simulink library "mssSimulink"  (R2024a)
settings: Solver=ode45  StartTime=0.0  StopTime=10.0  RelTol=1e-3
undefined symbols (not defined in the file): ABC, CN_data, CX_data, CY_data, D, G, Hoerner, K_supply, kt2ms, MA, magnitude, MRB, pathlength, RAO_Amp, RAO_Dir, RAO_Freq, RAO_Phase, RAO_Vel, RAO_yaw_back, RAO_yaw_quant, RAO_yaw_quantization_flag, rho_a, slcm, T_supply, table, vessel, vesselABC
libraries: $bdroot x99, simulink x13
(part 4 of 9)

== system mssSimulink/Modelling/Environmental Loads ==
  Force RAO : Subsystem  mask(Force RAO){RAO_Freq=vessel.forceRAO.w, RAO_Dir=vessel.headings, RAO_Vel=vessel.velocities, RAO_Amp=vessel.forceRAO.amp, RAO_Phase=vessel.forceRAO.phase, RAO_add_omega_0=on, RAO_add_omega_inf=on, RAO_yaw_quantization_flag=on, RAO_yaw_quant=10*pi/180, RAO_yaw_back=2.5*pi/180, RAO_speed_backlash_flag=on, RAO_speed_back=1, RAO_smoothing_flag=on}
      mask prompts: RAO_Freq "Vector of frequencies RAO_Freq (rad/s)"; RAO_Dir "Vector of directions RAO_Dir (rad)"; RAO_Vel "Vector of velocities RAO_Vel (m/s)"; RAO_Amp "6DOF Cell array with tables of Amplitudes RAO_Amp"; RAO_Phase "6DOF Cell array with tables of Phases RAO_Phase (rad)"; RAO_add_omega_0 "Add asymptotic RAO values for omega = 0"; RAO_add_omega_inf "Add asymptotic RAO values for omega = inf"; RAO_yaw_quantization_flag "LF estimator for yaw angle table lookup (backlash and quantization)"; RAO_yaw_quant "LF yaw angle quantization interval [rad]"; RAO_yaw_back "LF yaw angle backlash width [rad] (typically 1/4 of the quantization interval)"; RAO_speed_backlash_flag "Speed lookup backlash (avoid rapid speed data switching)"; RAO_speed_back "Speed backlash widht [m/s]"; RAO_smoothing_flag "Smooth the output to avoid switching transients due to table lookup"
      mask help:
      | Calculate the 6 degrees-of-freedom (DOF) wave-frequency excitation forces Tau_WF for a vessel from its Force Response Amplitude Operators (Force RAOs) and a sea state defined by a set of harmonic waves. The block takes the "Waves" bus from the MSS Waves block as input, as well as the vessel low-frequency (LF) motion in terms of the generalized position vector eta_LF and mean surge velocity U. See help for details.
      |
      | Copyright (C) NTNU 2005
      | Author: Oyvind N. Smogeli, 2005-05-03
      mask init:
      | % Add a second velocity if only one is given in order to avoid run-time errors in the table lookup blocks
      | if length(RAO_Vel) == 1
      | 
      | 	if RAO_Vel == 0 % Add a second identical data set for V = 5 m/s
      | 		RAO_Vel(2) = 5;
      | 	else % Add a second identical data set for V = 0 m/s
      | 		RAO_Vel = [0 RAO_Vel];
      | 	end
      | 
      | 	for dofno = 1:6
      | 		RAO_Amp{dofno}(:,:,2) = RAO_Amp{dofno}(:,:,1);
      | 		RAO_Phase{dofno}(:,:,2) = RAO_Phase{dofno}(:,:,1);
      | 	end
      | 
      | end
      | 
      | % Add RAO values for zero frequency: use values for lowest given frequency
      | if RAO_add_omega_0 > 0
      | 	
      | 	if min(RAO_Freq) > 0
      | 				
      | 		RAO_Freq = [0 RAO_Freq];
      | 		
      | 		for dofno = 1:6
      | 			RAO_Amp{dofno} = [RAO_Amp{dofno}(1,:,:); RAO_Amp{dofno}];
      | 			RAO_Phase{dofno} = [RAO_Phase{dofno}(1,:,:); RAO_Phase{dofno}];
      | 		end
      | 	
      | 	end
      | 	
      | end
      | 
      | % Add RAO values for high frequency: use values for highest given frequency
      | maxfreq = 100;
      | if RAO_add_omega_inf > 0
      | 
      | 	if max(RAO_Freq) < maxfreq
      | 			
      | 		newfreq = 2*max(RAO_Freq) - RAO_Freq(length(RAO_Freq)-1);
      | 		
      | 		RAO_Freq = [RAO_Freq newfreq maxfreq];
      | 		
      | 		for dofno = 1:6
      | 			RAO_Amp{dofno} = [RAO_Amp{dofno} ; zeros(2, length(RAO_Dir), length(RAO_Vel))];
      | 			RAO_Phase{dofno} = [RAO_Phase{dofno} ; zeros(2, length(RAO_Dir), length(RAO_Vel))];
      | 		end
      | 		
      | 	end
      | 
      | end
      mask Help:
      | <b>Part of the Marine Systems Simulator: MSS</b><br>
      | <br>
      | Calculate the 6 degrees-of-freedom (DOF) wave-frequency excitation forces Tau_WF
      | for a vessel from its Force Response Amplitude Operators (Force RAOs) and a sea
      | state defined by a set of harmonic waves. The block takes the &quot;Waves&quot; bus from
      | the MSS Waves block as input, as well as the vessel low-frequency (LF) motion in
      | terms of the generalized position vector eta_LF and mean surge velocity U.<p>The Force RAOs are defined in terms of a
      | vector of frequencies (RAO_Freq), a vector of directions (RAO_Dir), a vector of
      | velocities (RAO_Dir), a 6DOF cell array of 3D matrices with amplitudes
      | (RAO_Amp), and a 6DOF cell array of 3D matrices with phases (RAO_Phase), which
      | are all input in the block mask. The first dimension of the 3D matrices
      | corresponds to the frequencies, the second to the directions, and the third to
      | the velocities, such that e.g. the amplitude amp in heave (DOF #3) for frequency
      | number n_f, direction number n_d and velocity number n_v can be found from a =
      | RAO_Amp{3}(n_f, n_d, n_v).</p>
      | <p><b>Inputs:</b></p>
      | <p>Waves:&nbsp;&nbsp;&nbsp;&nbsp;&nbsp;&nbsp;&nbsp;&nbsp;&nbsp;&nbsp;&nbsp; Bus
      | containing the following signals<br>
      | &nbsp;&nbsp;&nbsp; Zeta_a:&nbsp;&nbsp;&nbsp;&nbsp;&nbsp;&nbsp;&nbsp; Vector of harmonic wave amplitudes [m]<br>
      | &nbsp;&nbsp;&nbsp; Omega:&nbsp;&nbsp;&nbsp;&nbsp;&nbsp;&nbsp; Vector of harmonic wave frequencies [rad/s]<br>
      | &nbsp;&nbsp;&nbsp; Phase:&nbsp;&nbsp;&nbsp;&nbsp;&nbsp;&nbsp;&nbsp;&nbsp; Vector of harmonic wave phases (random) [rad]<br>
      | &nbsp;&nbsp;&nbsp; Wavenum:&nbsp;&nbsp;&nbsp; Vector of harmonic wave numbers [1/m]<br>
      | &nbsp;&nbsp;&nbsp; Psi:&nbsp;&nbsp;&nbsp;&nbsp;&nbsp;&nbsp;&nbsp;&nbsp;&nbsp;&nbsp;&nbsp;&nbsp;&nbsp; Vector of harmonic wave directions [rad]</p>
      | <p>eta_LF:&nbsp;&nbsp;&nbsp;&nbsp;&nbsp;&nbsp;&nbsp;&nbsp;&nbsp;&nbsp;&nbsp;
      | Generalized 6DOF n-frame low-frequency position vector [x (m), y (m), z (m),
      | theta (rad), phi (rad), psi (rad)]<br>
      | U:&nbsp;&nbsp;&nbsp;&nbsp;&nbsp;&nbsp;&nbsp;&nbsp;&nbsp;&nbsp;&nbsp;&nbsp;&nbsp;&nbsp;&nbsp;&nbsp;&nbsp;&nbsp;&nbsp;
      | Low-frequency (mean) surge velocity&nbsp; [m/s]</p>
      | <p><b>Outputs:</b></p>
      | <p>tau_WF:&nbsp;&nbsp;&nbsp;&nbsp;&nbsp;&nbsp;&nbsp;&nbsp;&nbsp; Generalized
      | 6DOF h-frame force vector [X (N), Y (N), Z (N), K (Nm), M (Nm), N (Nm)]</p>
      | <p><b>Model validity:</b></p>
      | <p>The validity of the block is dependent on the validity of the given
      | RAO data set.</p>
      | <p>A proper RAO to be used with this block should contain at least 1 velocity, 5
      | directions (e.g. 0, 45, 90, 135 and 180 degrees) and 10-20 frequencies, for all
      | 6 DOF (surge, sway, heave, roll, pitch, yaw).</p>
      | <p>The block performs linear interpolation in frequencies and directions, and
      | uses the data set for the velocity closest to the input velocity (i.e. 'nearest'
      | interpolation in velocity). If the block recieves an input wave frequency or relative
      | wave direction outside the span of the data vectors RAO_Freq or RAO_Dir
      | respectively, the simulation stops and an error is returned. This means that a well-defined
      | RAO must contain data for both 0 and 180 degrees, and for frequencies covering
      | the desired range of wave frequencies. If desired, asymptotic values can be
      | automatically added for zero and infinity frequency to avoid runtime errors if
      | the wave freqeuncy exceeds the values in RAO_Freq (see checkboxes in the mask). </p>
      | <p>IMPORTANT NOTE: The RAO theory upon which this block is based is in reality
      | only valid when the vessel low-frequency (h-frame) motion is a constant surge
      | velocity only, and the vessel is performing wave-frequency oscillations about
      | the steadily translating h-frame.This means that the outputs from the block when
      | manoeuvering -- i.e. changing the surge velocity and/or yaw angle -- must be
      | interpreted with some care. A jump in the output must be expected when changing
      | between two velocity data sets, and frequency warping expected when changing the
      | yaw angle (due to interpolation in the phase). It is therefore recommended to
      | use backlash on the input velocity to avoid transient switching, and a quantized
      | yaw angle with backlash. The latter will lead to jump in the ouput when the yaw
      | angle changes from one quantized value to another, but will give better results
      | when keeping within one quantizer interval. The quantized yaw angle with
      | backlash and velocity with backlash are available as options via checkboxes in
      | the mask. If either of these are activated, proper values for the yaw
      | quantization interval, yaw backlash width, and the the speed backlash width
      | respectively must be set. Typical values could be a yaw quantization interval of
      | 5 degrees, yaw backlash width of 1/4-1/5 of the quantization interval, and speed
      | backlash width of 1 m/s. To avoid the most rapid transients when switching
      | between data sets, output smoothing is available as an option in the mask. If
      | this is enabled, the output during a transent is rate limited according to the
      | fastest recorded signal rate during normal operation.</p>
      | <p><b>Example mask input:</b></p><p>
      | As an example, the format of the mask input for 2 velocities, 3 directions and 5
      | frequencies is as follows:<p>RAO_Freq = [f1 f2 f3 f4 f5]<br>
      | RAO_Dir = [d1 d2 d3]<br>
      | RAO_Vel = [v1 v2]<p>Surge:<br>
      | RAO_Amp{1}(:,:,1)&nbsp; = [a1_111 a1_121 a1_131; a1_211 a1_221 a1_231; a1_311
      | a1_321 a1_331; a1_411 a1_421 a1_431; a1_511 a1_521 a1_531]<br>
      | RAO_Amp{1}(:,:,2)&nbsp; = [a1_112 a1_122 a1_132; a1_212 a1_222 a1_232; a1_312
      | a1_322 a1_332; a1_412 a1_422 a1_432; a1_512 a1_522 a1_532]<br>
      | RAO_Phase{1}(:,:,1) = [p1_111 p1_121 p1_131; p1_211 p1_221 p1_231; p1_311 p1_321
      | p1_331; p1_411 p1_421 p1_431; p1_511 p1_521 p1_531]<br>
      | RAO_Phase{1}(:,:,2) = [p1_112 p1_122 p1_132; p1_212 p1_222 p1_232; p1_312 p1_322
      | p1_332; p1_412 p1_422 p1_432; p1_512 p1_522 p1_532]<p>Sway:<br>
      | RAO_Amp{2}(:,:,1)&nbsp; = [a2_111 a2_121 a2_131; a2_211 a2_221 a2_231; a2_311
      | a2_321 a2_331; a2_411 a2_421 a2_431; a2_511 a2_521 a2_531]<br>
      | RAO_Amp{2}(:,:,2)&nbsp; = [a2_112 a2_122 a2_132; a2_212 a2_222 a2_232; a2_312
      | a2_322 a2_332; a2_412 a2_422 a2_432; a2_512 a2_522 a2_532]<br>
      | RAO_Phase{2}(:,:,1) = [p2_111 p2_121 p2_131; p2_211 p2_221 p2_231; p2_311 p2_321
      | p2_331; p2_411 p2_421 p2_431; p2_511 p2_521 p2_531]<br>
      | RAO_Phase{2}(:,:,2) = [p2_112 p2_122 p2_132; p2_212 p2_222 p2_232; p2_312 p2_322
      | p2_332; p2_412 p2_422 p2_432; p2_512 p2_522 p2_532]<p>...<p>Yaw:<br>
      | RAO_Amp{6}(:,:,1)&nbsp; = [a6_111 a6_121 a6_131; a6_211 a6_221 a6_231; a6_311
      | a6_321 a6_331; a6_411 a6_421 a6_431; a6_511 a6_521 a6_531]<br>
      | RAO_Amp{6}(:,:,2)&nbsp; = [a6_112 a6_122 a6_132; a6_212 a6_222 a6_232; a6_312
      | a6_322 a6_332; a6_412 a6_422 a6_432; a6_512 a6_522 a6_532]<br>
      | RAO_Phase{6}(:,:,1) = [p6_111 p6_121 p6_131; p6_211 p6_221 p6_231; p6_311 p6_321
      | p6_331; p6_411 p6_421 p6_431; p6_511 p6_521 p6_531]<br>
      | RAO_Phase{6}(:,:,2) = [p6_112 p6_122 p6_132; p6_212 p6_222 p6_232; p6_312 p6_322
      | p6_332; p6_412 p6_422 p6_432; p6_512 p6_522 p6_532]<p>where now for example the
      | amplitude and phase in sway (DOF 2) for frequency f5, direction d3 and velocity
      | v1 are given by RAO_Amp{2}(5,3,1) = a2_531 and RAO_Phase{2}(5,3,1) = p2_531.<p>
      | <b>Copyright (C) NTNU 2005</b></p>
      | <p><b>Author:</b> Oyvind N. Smogeli, 2005-05-03</p>
  Motion RAO : Subsystem  mask(Motion RAO){RAO_Freq=vessel.motionRAO.w, RAO_Dir=vessel.headings, RAO_Vel=vessel.velocities, RAO_Amp=vessel.motionRAO.amp, RAO_Phase=vessel.motionRAO.phase, RAO_add_omega_0=on, RAO_add_omega_inf=on, RAO_yaw_quantization_flag=off, RAO_yaw_quant=10*pi/180, RAO_yaw_back=2.5*pi/180, RAO_speed_backlash_flag=off, RAO_speed_back=2, RAO_smoothing_flag=on}
      mask prompts: RAO_Freq "Vector of frequencies RAO_Freq (rad/s)"; RAO_Dir "Vector of directions RAO_Dir (rad)"; RAO_Vel "Vector of velocities RAO_Vel (m/s)"; RAO_Amp "6DOF Cell array with tables of Amplitudes RAO_Amp"; RAO_Phase "6DOF Cell array with tables of Phases RAO_Phase (rad)"; RAO_add_omega_0 "Add asymptotic RAO values for omega = 0"; RAO_add_omega_inf "Add asymptotic RAO values for omega = inf"; RAO_yaw_quantization_flag "LF estimator for yaw angle table lookup (backlash and quantization)"; RAO_yaw_quant "LF yaw angle quantization interval [rad]"; RAO_yaw_back "LF yaw angle backlash width [rad] (typically 1/4 of the quantization interval)"; RAO_speed_backlash_flag "Speed lookup backlash (avoid rapid speed data switching)"; RAO_speed_back "Speed backlash widht [m/s]"; RAO_smoothing_flag "Smooth the output to avoid switching transients due to table lookup"
      mask help:
      | Calculate the wave-frequency motion of a vessel in 6 degrees-of-freedom (DOF) from its Motion Response Amplitude Operators (Motion RAOs) and a sea state defined by a set of harmonic waves. The block takes the "Waves" bus from the MSS Waves block as input, as well as the vessel low-frequency (LF) motion in terms of the generalized position vector eta_LF and mean surge velocity U. See help for details.
      |
      | Copyright (C) NTNU 2005
      | Author: Oyvind N. Smogeli, 2005-05-03
      mask init: same as mssSimulink/Modelling/Environmental Loads/Force RAO
      mask Help:
      | <b>Part of the Marine Systems Simulator: MSS</b><br>
      | <br>
      | Calculate the wave-frequency motion of a vessel in 6 degrees-of-freedom (DOF)
      | from its Motion Response Amplitude Operators (Motion RAOs) and a sea state
      | defined by a set of harmonic waves. The block takes the &quot;Waves&quot; bus from the MSS
      | Waves block as input, as well as the vessel low-frequency (LF) motion in terms
      | of the generalized position vector Eta_LF and surge velocity U.<p>
      | The Motion RAOs are defined in terms of a vector of frequencies (RAO_Freq), a
      | vector of directions (RAO_Dir), a vector of velocities (RAO_Dir), a 6DOF cell
      | array of 3D matrices with amplitudes (RAO_Amp), and a 6DOF cell array of 3D
      | matrices with phases (RAO_Phase), which are all input in the block mask. The
      | first dimension of the 3D matrices corresponds to the frequencies, the second to
      | the directions, and the third to the velocities, such that e.g. the amplitude
      | amp in heave (DOF #3) for frequency number n_f, direction number n_d and
      | velocity number n_v can be found from a = RAO_Amp{3}(n_f, n_d, n_v). </p>
      | <p><b>Inputs:</b></p>
      | <p>Waves:&nbsp;&nbsp;&nbsp;&nbsp;&nbsp;&nbsp;&nbsp;&nbsp;&nbsp;&nbsp;&nbsp; Bus
      | containing the following signals<br>
      | &nbsp;&nbsp;&nbsp; Zeta_a:&nbsp;&nbsp;&nbsp;&nbsp;&nbsp;&nbsp;&nbsp; Vector of harmonic wave amplitudes [m]<br>
      | &nbsp;&nbsp;&nbsp; Omega:&nbsp;&nbsp;&nbsp;&nbsp;&nbsp;&nbsp; Vector of harmonic wave frequencies [rad/s]<br>
      | &nbsp;&nbsp;&nbsp; Phase:&nbsp;&nbsp;&nbsp;&nbsp;&nbsp;&nbsp;&nbsp;&nbsp; Vector of harmonic wave phases (random) [rad]<br>
      | &nbsp;&nbsp;&nbsp; Wavenum:&nbsp;&nbsp;&nbsp; Vector of harmonic wave numbers [1/m]<br>
      | &nbsp;&nbsp;&nbsp; Psi:&nbsp;&nbsp;&nbsp;&nbsp;&nbsp;&nbsp;&nbsp;&nbsp;&nbsp;&nbsp;&nbsp;&nbsp;&nbsp; Vector of harmonic wave directions [rad]</p>
      | <p>eta_LF:&nbsp;&nbsp;&nbsp;&nbsp;&nbsp;&nbsp;&nbsp;&nbsp;&nbsp;&nbsp;&nbsp;
      | Generalized 6DOF n-frame low-frequency position vector [x (m), y (m), z (m),
      | theta (rad), phi (rad), psi (rad)]<br>
      | U:&nbsp;&nbsp;&nbsp;&nbsp;&nbsp;&nbsp;&nbsp;&nbsp;&nbsp;&nbsp;&nbsp;&nbsp;&nbsp;&nbsp;&nbsp;&nbsp;&nbsp;&nbsp;&nbsp;
      | Low-frequency (mean) surge velocity&nbsp; [m/s]</p>
      | <p><b>Outputs:</b></p>
      | <p>eta_WF:&nbsp;&nbsp;&nbsp;&nbsp;&nbsp;&nbsp;&nbsp;&nbsp;&nbsp; Generalized
      | 6DOF n-frame wave-frequency position vector [x (m), y (m), z (m), theta (rad),
      | phi (rad), psi (rad)]<br>
      | nu_WF:&nbsp;&nbsp;&nbsp;&nbsp;&nbsp;&nbsp;&nbsp;&nbsp;&nbsp;&nbsp; Generalized
      | 6DOF h-frame wave-frequency velocity vector [u (m/s), v (m/s), w (m/s), p
      | (rad/s), q (rad/s), r (rad/s)]<br>
      | nu_dot_WF:&nbsp;&nbsp;&nbsp;&nbsp; Generalized 6DOF h-frame wave-frequency
      | acceleration vector d/dt([u (m/s), v (m/s), w (m/s), p (rad/s), q (rad/s), r
      | (rad/s)])</p>
      | <p><b>Model validity:</b></p>
      | <p>The validity of the block is dependent on the validity of the given
      | RAO data set.</p>
      | <p>A proper RAO to be used with this block should contain at least 1 velocity, 5
      | directions (e.g. 0, 45, 90, 135 and 180 degrees) and 10-20 frequencies, for all
      | 6 DOF (surge, sway, heave, roll, pitch, yaw).</p>
      | <p>The block performs linear interpolation in frequencies and directions, and
      | uses the data set for the velocity closest to the input velocity (i.e. 'nearest'
      | interpolation in velocity). If the block recieves an input wave frequency or relative
      | wave direction outside the span of the data vectors RAO_Freq or RAO_Dir
      | respectively, the simulation stops and an error is returned. This means that a well-defined
      | RAO must contain data for both 0 and 180 degrees, and for frequencies covering
      | the desired range of wave frequencies. If desired, asymptotic values can be
      | automatically added for zero and infinity frequency to avoid runtime errors if
      | the wave freqeuncy exceeds the values in RAO_Freq (see checkboxes in the mask). </p>
      | <p>IMPORTANT NOTE: The RAO theory upon which this block is based is in reality
      | only valid when the vessel low-frequency (h-frame) motion is a constant surge
      | velocity only, and the vessel is performing wave-frequency oscillations about
      | the steadily translating h-frame.This means that the outputs from the block when
      | manoeuvering -- i.e. changing the surge velocity and/or yaw angle -- must be
      | interpreted with some care. A jump in the output must be expected when changing
      | between two velocity data sets, and frequency warping expected when changing the
      | yaw angle (due to interpolation in the phase). It is therefore recommended to
      | use backlash on the input velocity to avoid transient switching, and a quantized
      | yaw angle with backlash. The latter will lead to jump in the ouput when the yaw
      | angle changes from one quantizied value to another, but will give better results
      | when keeping within one quantizer interval. The quantized yaw angle with
      | backlash and velocity with backlash are available as options via checkboxes in
      | the mask. If either of these are activated, proper values for the yaw
      | quantization interval, yaw backlash width, and the the speed backlash width
      | respectively must be set. Typical values could be a yaw quantization interval of
      | 5 degrees, yaw backlash width of 1/4-1/5 of the quantization interval, and speed
      | backlash width of 1 m/s. To avoid the most rapid transients when switching
      | between data sets, output smoothing is available as an option in the mask. If
      | this is enabled, the output during a transent is rate limited according to the
      | fastest recorded signal rate during normal operation.</p>
      | <p><b>Example mask input:</b></p><p>
      | As an example, the format of the mask input for 2 velocities, 3 directions and 5
      | frequencies is as follows:<p>RAO_Freq = [f1 f2 f3 f4 f5]<br>
      | RAO_Dir = [d1 d2 d3]<br>
      | RAO_Vel = [v1 v2]<p>Surge:<br>
      | RAO_Amp{1}(:,:,1)&nbsp; = [a1_111 a1_121 a1_131; a1_211 a1_221 a1_231; a1_311
      | a1_321 a1_331; a1_411 a1_421 a1_431; a1_511 a1_521 a1_531]<br>
      | RAO_Amp{1}(:,:,2)&nbsp; = [a1_112 a1_122 a1_132; a1_212 a1_222 a1_232; a1_312
      | a1_322 a1_332; a1_412 a1_422 a1_432; a1_512 a1_522 a1_532]<br>
      | RAO_Phase{1}(:,:,1) = [p1_111 p1_121 p1_131; p1_211 p1_221 p1_231; p1_311 p1_321
      | p1_331; p1_411 p1_421 p1_431; p1_511 p1_521 p1_531]<br>
      | RAO_Phase{1}(:,:,2) = [p1_112 p1_122 p1_132; p1_212 p1_222 p1_232; p1_312 p1_322
      | p1_332; p1_412 p1_422 p1_432; p1_512 p1_522 p1_532]<p>Sway:<br>
      | RAO_Amp{2}(:,:,1)&nbsp; = [a2_111 a2_121 a2_131; a2_211 a2_221 a2_231; a2_311
      | a2_321 a2_331; a2_411 a2_421 a2_431; a2_511 a2_521 a2_531]<br>
      | RAO_Amp{2}(:,:,2)&nbsp; = [a2_112 a2_122 a2_132; a2_212 a2_222 a2_232; a2_312
      | a2_322 a2_332; a2_412 a2_422 a2_432; a2_512 a2_522 a2_532]<br>
      | RAO_Phase{2}(:,:,1) = [p2_111 p2_121 p2_131; p2_211 p2_221 p2_231; p2_311 p2_321
      | p2_331; p2_411 p2_421 p2_431; p2_511 p2_521 p2_531]<br>
      | RAO_Phase{2}(:,:,2) = [p2_112 p2_122 p2_132; p2_212 p2_222 p2_232; p2_312 p2_322
      | p2_332; p2_412 p2_422 p2_432; p2_512 p2_522 p2_532]<p>....<p>Yaw:<br>
      | RAO_Amp{6}(:,:,1)&nbsp; = [a6_111 a6_121 a6_131; a6_211 a6_221 a6_231; a6_311
      | a6_321 a6_331; a6_411 a6_421 a6_431; a6_511 a6_521 a6_531]<br>
      | RAO_Amp{6}(:,:,2)&nbsp; = [a6_112 a6_122 a6_132; a6_212 a6_222 a6_232; a6_312
      | a6_322 a6_332; a6_412 a6_422 a6_432; a6_512 a6_522 a6_532]<br>
      | RAO_Phase{6}(:,:,1) = [p6_111 p6_121 p6_131; p6_211 p6_221 p6_231; p6_311 p6_321
      | p6_331; p6_411 p6_421 p6_431; p6_511 p6_521 p6_531]<br>
      | RAO_Phase{6}(:,:,2) = [p6_112 p6_122 p6_132; p6_212 p6_222 p6_232; p6_312 p6_322
      | p6_332; p6_412 p6_422 p6_432; p6_512 p6_522 p6_532]<p>where now for example the
      | amplitude and phase in sway (DOF 2) for frequency f5, direction d3 and velocity
      | v1 are given by RAO_Amp{2}(5,3,1) = a2_531 and RAO_Phase{2}(5,3,1) = p2_531.<p>
      | <b>Copyright (C) NTNU 2005</b></p>
      | <p><b>Author:</b> Oyvind N. Smogeli, 2005-05-03</p></body>
  Utilities : Subsystem

== system mssSimulink/Modelling/Hydromecanics ==

== system mssSimulink/Modelling/Kinematics ==
  note: 3 DOF kinematic transformations
  note: 6 DOF kinematic transformations
  note: Euler angles
  note: Functions
  6 DOF transformation : Subsystem
  Crab angle : Subsystem
  Euler angles to inverse rotation matrix : Subsystem  mask(Rbn){}
      mask help:
      | Calculate the rotation matrix from NED coordinates to Body coordinates.
      |
      | Input: Theta = [phi, theta, psi]'
      |
      | Output: inv(Rzyx) (3x3)
      mask Help:
      | Calculate the rotation matrix from NED coordinates to Body coordinates.
      | 
      | Input: Theta = [phi, theta, psi]'
      | 
      | Output: inv(Rzyx) (3x3)
  Euler angles to rotation matrix : Subsystem  mask(Euler2R){}
      mask help: Determine the 3-by-3 rotation matrix from the Euler angles (roll, pitch, yaw) using the zyx convention.
      mask Display:
      | port_label('input',1,'theta')
      | port_label('output',1,'R')
  Euler angles to attitude transformation matrix : Subsystem  mask(Euler2T){}
      mask help: Determine the 3-by-3 attitude transformation matrix from the Euler angles (roll, pitch, yaw).
      mask Display:
      | port_label('input',1,'theta')
      | port_label('output',1,'T')
  "Rotation matrix in yaw " : Subsystem
      mask help:
      | b = R(psi)* a
      |
      | where
      |
      | input 1:    psi
      | input 2:    a - vector dim 3
      | output 1:  b - vector dim 3
      mask Display:
      | port_label('output', 1, 'R(psi)*v')
      | port_label('input', 1, 'psi')
      | port_label('input', 2, 'v')
  Transformation of generalized force : Subsystem  mask(Transformation of generalized force){}
      mask help:
      | Transforms a generalized force vector from one coordinate to a
      | new coordinate.
      |
      | Takes the force vector in one point and the vector to the new point
      | as input, and gives the force vector in the new point as output.
      |
      | Uses a Simulink version of the Hmtrx (inversed and transposed) gnc
      | matlab function.
  Transformation of generalized velocity : Subsystem  mask(Velocity transformation){}
      mask help:
      | Transforms a generalized velocity vector from one coordinate to a
      | new coordinate.
      |
      | Takes the velocity vector in one point and the vector to the new point
      | as input, and gives the velocity vector in the new point as output.
      |
      | Uses a Simulink version of the Hmtrx gnc matlab function.
      mask Help:
      | Transforms a generalized velocity vector from one coordinate to a
      | new coordinate.
      | 
      | Takes the velocity vector in one point and the vector to the new point
      | as input, and gives the velocity vector in the new point as output.
      | 
      | Uses a Simulink version of the Hmtrx gnc matlab function.
  Transposed rotation matrix in yaw : Subsystem
      mask help:
      | b = R'(psi)* a
      |
      | where
      |
      | input 1:    psi
      | input 2:    a - vector dim 3
      | output 1:  b - vector dim 3
      mask Display:
      | port_label('output', 1, 'R''(psi)*v')
      | port_label('input', 1, 'psi')
      | port_label('input', 2, 'v')

== system mssSimulink/Modelling/Kinetics  ==
  3 DOF Eqs. of motion : Subsystem  mask(Equations of motion){CoriolisOnOff=on, nu0=[0 0 0], eta0=[0 0 0]}
      mask prompts: CoriolisOnOff "Coriolis and centripetal forces (check box to turn on)"; nu0 "Initial velocities (u,v,r)"; eta0 "Initial position/attitude (x,y,psi)"
      mask help:
      | 3 DOF equations of motion (surge, sway, roll and pitch)
      |
      |    eta_dot = J(eta)*nu
      |    (M_RB+M_A)*nu_dot + C_RB(nu)nu+C_A(nu_r)nu_r  =  tau
      |
      |    nu_r = nu-nu_c    (relative velocity)
      |    nu_c = [u_c, v_c, 0]  slowly-varying current velocity
      |
      | where nu = [u,v,r]' and eta = [x,y,psi]'
      |
      | The Coriolis and centripetal matrix C(nu) is computed automatically using the system inertia matrix M and nu,  see Chapter 3 in Fossen (2002) for details.
      |
      | T. I. Fossen (2002). Marine Control Systems: Guidance, Navigation and Control of Ships, Rigs and Underwater Vehicles, Marine Cybernetics AS, ISBN 82-92356-00-2
  6 DOF Eqs. of motion : Subsystem  mask(Equations of motion){CoriolisOnOff=on, nu0=[0 0 0 0 0 0], eta0=[0 0 0 0 0 0]}
      mask prompts: CoriolisOnOff "Coriolis and centripetal forces (check box to turn on)"; nu0 "Initial velocities (u,v,w,p,q,r)"; eta0 "Initial position/attitude (x,y,z,phi,theta,psi)"
      mask help:
      | 6 DOF equations of motion (surge, sway, heave, roll, pitch and yaw)
      |
      |    eta_dot = J(eta)*nu
      |    (M_RB+M_A)*nu_dot + C_RB(nu)nu+C_A(nu_r)nu_r  =  tau
      |
      |    nu_r = nu-nu_c    (relative velocity)
      |    nu_c = [u_c,v_c,w_c,0,0,0]  slowly-varying current velocity
      |
      | where nu = [u,v,w,p,q,r]'  and eta = [x,y,x,phi,theta,psi]'
      |
      | The Coriolis and centripetal matrix C(nu) is computed automatically using the system inertia matrix M and nu,  see Chapter 3 in Fossen (2002) for details.
      |
      | T. I. Fossen (2002). Marine Control Systems: Guidance, Navigation and Control of Ships, Rigs and Underwater Vehicles, Marine Cybernetics AS, ISBN 82-92356-00-2
  Support : Subsystem

== system mssSimulink/Modelling/Propulsion ==
  Actuator Configuration : Subsystem
  Open-water propeller characteristics : Subsystem  mask(Open-water propeller characteristics){Par_Thruster_D=1, Par_Thruster_Ktp=[-0.1060 -0.3246 0.4594], Par_Thruster_Kqp=[-0.0186 -0.0399 0.0680], Par_Thruster_reverse_reduction=0.8, Glob_rhow=1025}
      mask prompts: Par_Thruster_D "Thruster diameter [m]"; Par_Thruster_Ktp "Kt polynomial Ktp"; Par_Thruster_Kqp "Kq polynomial Kqp"; Par_Thruster_reverse_reduction "Reverse direction thrust reduction factor [-]"; Glob_rhow "Density of seawater [kg/m^3]"
      mask help:
      | Calculate the thrust and torque of a fixed pitch propeller, based on a polynomial representation of thrust and torque coefficients Kt and Kq from the open-water characteristics. Kt and Kq are defined as polynomials Ktp and Kqp in the advance number J=Va/(nD):
      |
      | Kt = Ktp(1)*J^2 + Kqp(2)*J + Kqp(3)
      | Kq = Kqp(1)*J^2 + Kqp(2)*J + Kqp(3)
      |
      | where n is the shaft speed, D the propelelr diameter and Va the advance velocity of the propeller. The relationship between the thrust T and torque Q and the coefficients Kt and Kq is:
      |
      | T = Kt*rho*D^4
      | Q = Kq*rho*D^5
      |
      | where rho is the density of water. See help for details.
      |
      | Copyright (C) 2005 NTNU
      |
      | Author: Oyvind Notland Smogeli
      mask Help:
      | <p>
      | <b>Part of the Marine Systems Simulator: MSS</b></p>
      | <p>Calculate the thrust and torque of a fixed pitch propeller, based on a polynomial
      | representation of thrust and torque coefficients from the open-water
      | characteristics.</p>
      | <p><b>Inputs: </b> </p>
      | <p>n: [1/s] Propeller shaft speed<br>
      | Va: [m/s] Propeller advance speed</p>
      | <p><b>Outputs: </b> </p>
      | <p>T: [N] Propeller thrust<br>
      | Q: [Nm] Propeller torque<p><b>Model validity:</b><p>The model gives the thrust and torque from a polynomial of the form:<p>T = sign(n)*[T_nn*n^2 + T_Vn*Va*n + T_VV*Va^2]<br>Q = sign(n)*[Q_nn*n^2 + Q_Vn*Va*n + Q_VV*Va^2]<p>If the expression in brackets becomes negative, it is set to zero.
      | Propeller windmilling is therefore not accounted for.
      | The thrust is modified by a reduction factor when the thruster is
      | reversed (n &lt; 0), and the torque kept unmodified. Negative advance velocities
      | are treated as zero.<p>The coefficients are:<p>T_nn = Ktp(3)*rhow*D^4<br>T_Vn = Ktp(2)*rhow*D^3<br>T_VV = Ktp(1)*rhow*D^2<br>Q_nn = Kqp(3)*rhow*D^5<br>Q_Vn = Kqp(2)*rhow*D^4<br>Q_VV = Kqp(1)*rhow*D^3<p>
      | where rhow is the density of seawater, D the propeller diameter, and
      | Ktp and Kqp are the polynomials defined in the mask:<p>Kt = Ktp(1)*J^2 + Kqp(2)*J + Kqp(3)<br>Kq = Kqp(1)*J^2 + Kqp(2)*J + Kqp(3)<p>where J is the advance number, J = Va/(n*D).
      | The relationship between the thrust and torque and the coefficients Kt and Kq
      | is:<p>T = Kt*rhow*D^4<br>Q = Kq*rhow*D^5<p>Example input data for a
      | Wageningen B-series propeller with pitch ratio P/D = 1, number of blades Z = 4 and
      | expanded blade area ratio EAR = 0.7:<p>Ktp = [-0.1060 -0.3246 0.4594]<br>Kqp = [-0.0186 -0.0399 0.0680]<br>
      | reverse_reduction = 0.8<p>
      | <b>Copyright NTNU 2005</b></p>
      | <p><b>Author:</b> Oyvind N. Smogeli, 2005-05-03</p>
      mask Display:
      | image(imread('simulink/figs/propeller.jpg'))
      | port_label('input', 1, 'n [1/s]')
      | port_label('input', 2, 'Va [m/s]')
      | port_label('output', 1, 'T [N]')
      | port_label('output', 2, 'Q [Nm]')
  Propeller shaft dynamics : Subsystem  mask(Propeller){rpm_max=.5, rpm_rate=.5, tc=1}
      mask prompts: rpm_max "Max RPM:"; rpm_rate "Max RPM Rate:"; tc "Time Constant (sec):"
      mask help:
      | Integrator in a feedback loop with rate and magnitude saturation. When the system does not saturate, it behaves as a first order system with  the time constant entered in the mask
      | Copyright (C) 2005 NTNU
      | Author: T.I. Fossen

== system mssSimulink/Navigation/Estimators ==
  Discerte-time EKF for SOG and COG : Subsystem  InitFcn=|  mask{alpha_1=0.00001, alpha_2=0.00001, Qd=100*diag([0.1,0.1]), Rd=0.1*diag([1 1]), h_samp=0.2}
      | clear x_prd;
      | clear P_prd;
      mask prompts: alpha_1 "alpha_1 - Singer constant SOG"; alpha_2 "alpha_2 Singer constant COG"; Qd "Qd - Discrete-time process covariance matrix"; Rd "Rd - Discrete-time measurement covariance matrix"; h_samp "h_samp - Sampling time of position measurements (seconds)"
      mask DialogControl DescTextVar Prompt: This function estimates the SOG, COG, and course rate from positions measurements (x, y) expressed  in NED using the 5-state discrete-time EKF of Fossen and Fossen (2021). The states estimated include positions (x, y),  SOG (U), COG (chi), and course rate (omega_chi) in the NED coordinate system.
  Kalman filter based autopilot wave filter : Subsystem  mask{lambda=0.1, w_o=1.0, T_b=1000, K=0.1, T=100, r=1, q1=100, q2=0.01, q3=0.01, P0=1*eye(5)}
      mask prompts: lambda "Relative damping ratio of wave spectrum: lambda"; w_o "Peak frequency of wave spectrum: w_o (rad/s)"; T_b "Bias time constant: T_b (s)"; K "Nomoto gain constant: K (1/s)"; T "Nomoto time constant: T (s)"; r "Compass variance: r"; q1 "Wave model variance: q1"; q2 "Ship model variance: q2"; q3 "Bias model variance: q3"; P0 "Initial covariance matrix"
      mask Display: disp('Only\n Compass')
  Passive DP wave filter : Subsystem  mask{lambda=0.1*diag([1 1 1]), w_o=diag([0.8 0.8 0.8]), K4=0.1*diag([1 1 0.1]), K3=0.1*diag([1 1 0.1]), w_c=1.3*diag([0.8 0.8 0.8]), T_b=diag([100 100 100]), M=diag([1 1 1]), D=diag([1 1 1])}
      mask prompts: lambda "Relative damping ratio of wave spectrum: lambda"; w_o "Peak frequency of wave spectrum: w_o (rad/s)"; K4 "Velocity observer gain: K4"; K3 "Bias observer gain: K3"; w_c "Filter cut-off frequency: w_c (rad/s)"; T_b "Bias time constants: T_b (s)"; M "system inertia matrix: M"; D "linear damping matrix: D"
      mask Display: disp('GPS and\n Gyro')
  Passive autopilot wave filter 1 : Subsystem  mask(wave spectrum damping ratio){lambda=0.1, w_o=1.2, K4=0.1, K5=0.01, w_c=1.3, T=100, K=1, T_b=100}
      mask prompts: lambda "Relative damping ratio of wave spectrum: lambda"; w_o "Peak frequency of wave spectrum: w_o (rad/s)"; K4 "Yaw rate observer gain: K4"; K5 "Bias observer gain: K5"; w_c "Filter cut-off frequency: w_c (rad/s)"; T "Nomoto time constant: T (s)"; K "Nomoto gain: K (1/s)"; T_b "Rudder bias time constant: T_b (s)"
      mask Display: disp('Only\n Compass')
  Passive autopilot wave filter 2 : Subsystem  mask(wave spectrum damping ratio){lambda=0.1, w_o=1.2, K4=0.1, zeta_n=0.01, w_c=2, T_b=100}
      mask prompts: lambda "Relative damping ratio of wave spectrum: lambda"; w_o "Peak frequency of wave spectrum: w_o (rad/s)"; K4 "Bias observer gain: K4"; zeta_n "Relative damping ratio in gyro notch filter: zeta_n"; w_c "Filter cut-off frequency: w_c (rad/s)"; T_b "Bias time constant: T_b (s)"
      mask Display: disp('Compass\n and Gyro')

== system mssSimulink/Navigation/Sensors  ==

== system mssSimulink/Utilities/Dynamics ==
  2nd order time constant : Subsystem  mask(2nd order time constant){T=3}
      mask prompts: T "Time constant [s]"
      mask help: Approximate 2nd order time constnant, implemented as a second order system with damping ratio 1 and eigenfrequency w = 1.5/T, where T is the time constant.

== system mssSimulink/Utilities/Math Operations ==
  Unit Conversion : Subsystem  mask(Unit Conversion){in=deg2rad}
      mask prompts: in "Convert"
      mask help:
      | Block to convert units. If the input in is a vector,
      | all the components are converted using the same conversion factor.
      |
      | Copyright (C) 2005 NTNU
      | Author:  Tristan Perez
      mask init:
      | if  in==1,
      | k=pi/180;
      | elseif  in==2,
      | k=180/pi;
      | elseif in==3,
      | k = .5145;
      | elseif in ==4,
      | k = 1/.5145;
      | 
      | end
      mask TypeOptions in: deg2rad | rad2deg | kt2m/sec | m/sec2 kt
  "[-inf inf] to [-pi pi]" : Subsystem  mask([-inf inf] to [-pi pi]){}
      mask help: Converts an angle in rad to (-pi pi)
  "[-pi pi] to [-inf inf]" : Subsystem  mask([-pi pi] to [-inf inf]){}
      mask help: Maps an angle in the range [-pi pi] to the range [-inf inf].
  deg to 180/180 : Subsystem  mask(deg to 180/180){}
      mask help: Converts an angle in deg to +- 180 deg
      mask Display: disp('[0 360] to [-180 180]')
  ssa : Subsystem

== system mssSimulink/Utilities/Simulation tools ==
  6DOF comparison : Subsystem  mask(6DOF comparison){}
      mask help: Compare two 6DOF signals (i.e. motion or force). To view the signals, open the scope inside the block.
  Signal range error : Subsystem  mask(Signal range error){Values=[-3 -1], message=Test message}
      mask prompts: Values "Vector spanning the allowed input signal range"; message "Error message"
      mask help:
      | Stop the simulation and return a user specified error message if any of the values in the input signal is outside the range spanned by the vector specified in the mask. The sizes of the input vector and mask vector are arbitrary, the allowed signal range is taken as the max and min values of the vector in the mask.
      |
      | Author: Oyvind Notland Smogeli, 2005-05-15
  Stop simulation : S-Function  FunctionName=stopSimulation  Parameters=message  SFunctionDeploymentMode=off  EnableBusSupport=off  mask(Stop simulation){message='Error message test'}
      mask prompts: message "Error message (string)"
      mask help:
      | Stop the simulation and return a user specified error message if the input signal is outside the range [0, 1>
      |
      | Author: Oyvind Notland Smogeli, 2005-05-13
      mask Display: port_label('input', 1, '')

== system mssSimulink/Utilities/Visualization ==
  North-East plot : Subsystem  StopFcn=|  mask{decimation=100}
      | x = xyplot.Data(:,1);
      | y = xyplot.Data(:,2);
      | wptX = waypoints(:,1);
      | wptY = waypoints(:,2);
      | figure(gcf);
      | plot(y,x,'b','linewidth',2);
      | hold on;
      | plot(wptY,wptX,'o','MarkerSize',15,'MarkerEdgeColor','k','MarkerFaceColor','c');
      | hold off;
      | xlabel('East (m)', 'FontSize', 14);
      | ylabel('North (m)', 'FontSize', 14);
      | title('North-East Positions (m)', 'FontSize', 14);
      | axis('equal');
      | grid;
  "North-East plot  " : Subsystem  StopFcn=|  mask{decimation=100}
      | x = xyplot.Data(:,1);
      | y = xyplot.Data(:,2);
      | figure(gcf);
      | plot(y,x,'b','linewidth',2);
      | xlabel('East (m)', 'FontSize', 14);
      | ylabel('North (m)', 'FontSize', 14);
      | title('North-East Positions (m)', 'FontSize', 14);
      | axis('equal');
      | grid;

== system mssSimulink/Control/Autopilots/Course autopilot ==
  "chi_d " : Inport
  omega_chi_d : Inport  Port=2
  chi : Inport  Port=3
  omega_chi : Inport  Port=4
  Integrator : Integrator
  Kd : Gain  Gain=m*(2*zeta*wn-1/T_nomoto)  SaturateOnIntegerOverflow=on  OutDataTypeStr=Inherit: Same as input  ParamDataTypeStr=Inherit: Same as input
  Ki : Gain  Gain=m*wn^3/10  SaturateOnIntegerOverflow=on  OutDataTypeStr=Inherit: Same as input  ParamDataTypeStr=Inherit: Same as input
  Kp : Gain  Gain=m*wn^2  SaturateOnIntegerOverflow=on  OutDataTypeStr=Inherit: Same as input  ParamDataTypeStr=Inherit: Same as input
  Sum1 : Sum  Inputs=+++  InputSameDT=on  SaturateOnIntegerOverflow=on  OutDataTypeStr=Inherit: Same as first input
  Sum2 : Sum  Inputs=|+-  InputSameDT=on  SaturateOnIntegerOverflow=on  OutDataTypeStr=Inherit: Same as first input
  Sum3 : Sum  Inputs=|-+  InputSameDT=on  SaturateOnIntegerOverflow=on  OutDataTypeStr=Inherit: Same as first input
  Sum4 : Sum  Inputs=++|  InputSameDT=on  SaturateOnIntegerOverflow=on  OutDataTypeStr=Inherit: Same as first input
  m/T_Nomoto : Gain  Gain=m/T_nomoto  SaturateOnIntegerOverflow=on  OutDataTypeStr=Inherit: Same as input  ParamDataTypeStr=Inherit: Same as input
  "ssa " : $bdroot/Utilities/Math Operations/ssa  SystemSampleTime=-1  VariantActivationTime=update diagram  AllowFlexibleInterface=on  Latency=0  AutoFrameSizeCalculation=off
  tau_N : Outport
  wires:
  Kd/1 -> Sum1/1
  omega_chi/1 -> Sum3/1
  chi/1 -> Sum2/2
  "chi_d "/1 -> Sum2/1
  Sum2/1 -> "ssa "/1
  Sum1/1 -> Sum4/2  "tau_PID"
  "ssa "/1 -> Ki/1, Kp/1
  Ki/1 -> Integrator/1
  Integrator/1 -> Sum1/3
  Sum3/1 -> Kd/1
  omega_chi_d/1 -> Sum3/2, m/T_Nomoto/1
  Sum4/1 -> tau_N/1
  m/T_Nomoto/1 -> Sum4/1  "tau_FF"
  Kp/1 -> Sum1/2  "tau_PID"

== system mssSimulink/Control/Autopilots/Course autopilot  ==
  chi_d : Inport
  omega_chi_d : Inport  Port=2
  chi : Inport  Port=3
  omega_chi : Inport  Port=4
  D-action : Gain  Gain=Kp*Td  SaturateOnIntegerOverflow=on  OutDataTypeStr=Inherit: Same as input  ParamDataTypeStr=Inherit: Same as input
  D-action2 : Gain  Gain=1/K_nomoto  SaturateOnIntegerOverflow=on  OutDataTypeStr=Inherit: Same as input  ParamDataTypeStr=Inherit: Same as input
  "I-action " : Gain  Gain=1/Ti  SaturateOnIntegerOverflow=on  OutDataTypeStr=Inherit: Same as input  ParamDataTypeStr=Inherit: Same as input
  Integral : TransferFcn  Denominator=[1 0]
  P-action : Gain  Gain=Kp  SaturateOnIntegerOverflow=on  OutDataTypeStr=Inherit: Same as input  ParamDataTypeStr=Inherit: Same as input
  Sum1 : Sum  Inputs=++++  InputSameDT=on  SaturateOnIntegerOverflow=on  OutDataTypeStr=Inherit: Same as first input
  Sum2 : Sum  Inputs=|+-  InputSameDT=on  SaturateOnIntegerOverflow=on  OutDataTypeStr=Inherit: Same as first input
  Sum3 : Sum  Inputs=|+-  InputSameDT=on  SaturateOnIntegerOverflow=on  OutDataTypeStr=Inherit: Same as first input
  "ssa " : $bdroot/Utilities/Math Operations/ssa  SystemSampleTime=-1  VariantActivationTime=update diagram  AllowFlexibleInterface=on  Latency=0  AutoFrameSizeCalculation=off
  tau_N : Outport  InitialOutput=0  VectorParamsAs1DForOutWhenUnconnected=off
  wires:
  chi_d/1 -> Sum2/1
  "ssa "/1 -> P-action/1
  Sum2/1 -> "ssa "/1
  D-action2/1 -> Sum1/4
  omega_chi_d/1 -> D-action2/1, Sum3/1
  omega_chi/1 -> Sum3/2
  chi/1 -> Sum2/2
  Sum3/1 -> D-action/1
  Integral/1 -> Sum1/2
  Sum1/1 -> tau_N/1
  D-action/1 -> Sum1/3
  "I-action "/1 -> Integral/1
  P-action/1 -> Sum1/1, "I-action "/1

== system mssSimulink/Control/Autopilots/Heading autopilot ==
  psi_d : Inport
  r_d : Inport  Port=2
  d/dt(r_d) : Inport  Port=3
  psi : Inport  Port=4
  r : Inport  Port=5
  D-action : Gain  Gain=Kp*Td  SaturateOnIntegerOverflow=on  OutDataTypeStr=Inherit: Same as input  ParamDataTypeStr=Inherit: Same as input
  D-action1 : Gain  Gain=T_nomoto  SaturateOnIntegerOverflow=on  OutDataTypeStr=Inherit: Same as input  ParamDataTypeStr=Inherit: Same as input
  D-action2 : Gain  Gain=1/K_nomoto  SaturateOnIntegerOverflow=on  OutDataTypeStr=Inherit: Same as input  ParamDataTypeStr=Inherit: Same as input
  "I-action " : Gain  Gain=1/Ti  SaturateOnIntegerOverflow=on  OutDataTypeStr=Inherit: Same as input  ParamDataTypeStr=Inherit: Same as input
  Integral : TransferFcn  Denominator=[1 0]
  P-action : Gain  Gain=Kp  SaturateOnIntegerOverflow=on  OutDataTypeStr=Inherit: Same as input  ParamDataTypeStr=Inherit: Same as input
  Sum1 : Sum  Inputs=++++  InputSameDT=on  SaturateOnIntegerOverflow=on  OutDataTypeStr=Inherit: Same as first input
  Sum2 : Sum  Inputs=|+-  InputSameDT=on  SaturateOnIntegerOverflow=on  OutDataTypeStr=Inherit: Same as first input
  Sum3 : Sum  Inputs=|+-  InputSameDT=on  SaturateOnIntegerOverflow=on  OutDataTypeStr=Inherit: Same as first input
  Sum4 : Sum  Inputs=|++  InputSameDT=on  SaturateOnIntegerOverflow=on  OutDataTypeStr=Inherit: Same as first input
  "ssa " : $bdroot/Utilities/Math Operations/ssa  SystemSampleTime=-1  VariantActivationTime=update diagram  AllowFlexibleInterface=on  Latency=0  AutoFrameSizeCalculation=off
  tau_N : Outport  InitialOutput=0  VectorParamsAs1DForOutWhenUnconnected=off
  wires:
  P-action/1 -> "I-action "/1, Sum1/1
  "I-action "/1 -> Integral/1
  D-action/1 -> Sum1/3
  Sum1/1 -> tau_N/1
  Integral/1 -> Sum1/2
  Sum3/1 -> D-action/1
  psi/1 -> Sum2/2
  d/dt(r_d)/1 -> D-action1/1
  r/1 -> Sum3/2
  r_d/1 -> Sum3/1, Sum4/1
  D-action1/1 -> Sum4/2
  Sum4/1 -> D-action2/1
  D-action2/1 -> Sum1/4
  Sum2/1 -> "ssa "/1
  "ssa "/1 -> P-action/1
  psi_d/1 -> Sum2/1

== system mssSimulink/Control/DP/Nonlinear PID ==
  eta_ref : Inport
  eta : Inport  Port=2
  nu : Inport  Port=3
  Demux : Demux  Outputs=3
  Integrator : Integrator
  Kd : Gain  Gain=Kd  Multiplication=Matrix(K*u)  SaturateOnIntegerOverflow=on  OutDataTypeStr=Inherit: Same as input  ParamDataTypeStr=Inherit: Same as input
  Ki : Gain  Gain=Ki  Multiplication=Matrix(K*u)  SaturateOnIntegerOverflow=on  OutDataTypeStr=Inherit: Same as input  ParamDataTypeStr=Inherit: Same as input
  Kp : Gain  Gain=Kp  Multiplication=Matrix(K*u)  SaturateOnIntegerOverflow=on  OutDataTypeStr=Inherit: Same as input  ParamDataTypeStr=Inherit: Same as input
  Mux : Mux  Inputs=3
  Sum1 : Sum  Inputs=|+-  InputSameDT=on  SaturateOnIntegerOverflow=on  OutDataTypeStr=Inherit: Same as first input
  Sum2 : Sum  Inputs=+-|  InputSameDT=on  SaturateOnIntegerOverflow=on  OutDataTypeStr=Inherit: Same as first input
  Sum3 : Sum  Inputs=|++  InputSameDT=on  SaturateOnIntegerOverflow=on  OutDataTypeStr=Inherit: Same as first input
  "Transposed rotation matrix in yaw " : $bdroot/Modelling/Kinematics/Transposed rotation  matrix in yaw
  "ssa " : $bdroot/Utilities/Math Operations/ssa  SystemSampleTime=-1  VariantActivationTime=update diagram  AllowFlexibleInterface=on  Latency=0  AutoFrameSizeCalculation=off
  yaw angle : Fcn  Expr=u(3)
  tau : Outport  InitialOutput=0  VectorParamsAs1DForOutWhenUnconnected=off
  wires:
  "Transposed rotation matrix in yaw "/1 -> Kp/1, Integrator/1
  Ki/1 -> Sum3/2
  Sum3/1 -> Sum1/1
  Kp/1 -> Sum3/1
  Integrator/1 -> Ki/1
  Kd/1 -> Sum1/2
  nu/1 -> Kd/1
  eta/1 -> yaw angle/1, Sum2/2
  Sum1/1 -> tau/1
  eta_ref/1 -> Sum2/1
  Demux/3 -> "ssa "/1
  Sum2/1 -> Demux/1  "regulation error"
  "ssa "/1 -> Mux/3
  Demux/2 -> Mux/2
  Demux/1 -> Mux/1
  Mux/1 -> "Transposed rotation matrix in yaw "/2
  yaw angle/1 -> "Transposed rotation matrix in yaw "/1  "psi"

== system mssSimulink/Environment/Current/North-East current ==
  beta_c (deg) : Inport
  V_c (m/s) : Inport  Port=2
  Gain : Gain  Gain=pi/180
  Mux : Mux  Inputs=6
  Product : Product  RndMeth=Zero
  Product1 : Product  RndMeth=Zero
  cos : Trigonometry  Operator=cos
  sin : Trigonometry
  zero : Constant  Value=0
  nu_c : Outport  VectorParamsAs1DForOutWhenUnconnected=off
  wires:
  Gain/1 -> sin/1, cos/1
  cos/1 -> Product/1
  V_c (m/s)/1 -> Product1/2, Product/2
  sin/1 -> Product1/1
  Product/1 -> Mux/1
  Product1/1 -> Mux/2
  zero/1 -> Mux/3, Mux/4, Mux/5, Mux/6
  beta_c (deg)/1 -> Gain/1
  Mux/1 -> nu_c/1

== system mssSimulink/Environment/Waves/ Gaussian Random Process ==
  In1 : Inport
  "Amp Reg Comp. " : Constant  Value=areg  VectorParams1D=off
  Dot Product : DotProduct  OutDataTypeStr=Inherit: Inherit via internal rule
  Freq1 : Constant  Value=freq  VectorParams1D=off
  Model Info1 : simulink/Model-Wide Utilities/Model Info  Frame=on  DisplayStringWithTags=|  HorizontalTextAlignment=Center  LeftAlignmentValue=0.5
      | Fourier Representation of a Gaussian Random Process
      | (C) Copyright 2004 Tristan Perez
  Product : Product  SaturateOnIntegerOverflow=on  OutDataTypeStr=Inherit: Same as first input
  Random Phases1 : Constant  Value=phases  VectorParams1D=off
  Sum : Sum  Inputs=|++  SaturateOnIntegerOverflow=on
  Trigonometric Function : Trigonometry  Operator=cos
  Out : Outport  VectorParamsAs1DForOutWhenUnconnected=off
  wires:
  Trigonometric Function/1 -> Dot Product/2
  Sum/1 -> Trigonometric Function/1
  Dot Product/1 -> Out/1
  In1/1 -> Product/2
  Freq1/1 -> Product/1
  Product/1 -> Sum/1
  Random Phases1/1 -> Sum/2
  "Amp Reg Comp. "/1 -> Dot Product/1

== system mssSimulink/Environment/Waves/Encounter frequency correction ==
  Waves : Inport
  U : Inport  Port=2
  Psi : Inport  Port=3
  Bus Creator : BusCreator  Inputs=5
  Bus Selector : BusSelector  OutputSignals=Omega,Psi,Zeta_a,Wavenum,Phase
  Sum : Sum  Inputs=|+-
  Terminator : Terminator
  W_wave 2 W_enc (no absolute value) : $bdroot/Environment/Waves/W_wave 2 W_enc (no absolute value)
  "Waves " : Outport  VectorParamsAs1DForOutWhenUnconnected=off
  wires:
  W_wave 2 W_enc (no absolute value)/2 -> Bus Creator/4  "Wavenum"
  Bus Creator/1 -> "Waves "/1
  W_wave 2 W_enc (no absolute value)/1 -> Bus Creator/1  "Omega"
  Psi/1 -> Sum/2
  Bus Selector/5 -> Bus Creator/5  "<Phase>"
  Bus Selector/4 -> Terminator/1  "<Wavenum>"
  Bus Selector/3 -> Bus Creator/3  "<Zeta_a>"
  Waves/1 -> Bus Selector/1
  Bus Selector/2 -> Bus Creator/2, Sum/1  "<Psi>"
  Sum/1 -> W_wave 2 W_enc (no absolute value)/3
  U/1 -> W_wave 2 W_enc (no absolute value)/1
  Bus Selector/1 -> W_wave 2 W_enc (no absolute value)/2  "<Omega>"

== system mssSimulink/Environment/Waves/Linear 2nd-order wave spectrum ==
  white noise : Inport
  Linear 2nd-order wave spectrum : TransferFcn  Numerator=[2*lambda*w_0*sigma 0]  Denominator="[1 2*lambda*w_0  w_0^2]"
  wave amplitude : Outport  VectorParamsAs1DForOutWhenUnconnected=off
  wires:
  Linear 2nd-order wave spectrum/1 -> wave amplitude/1
  white noise/1 -> Linear 2nd-order wave spectrum/1

== system mssSimulink/Environment/Waves/W_wave 2 W_enc (no absolute value) ==
  U : Inport
  "W " : Inport  Port=2
  "Enc. Angle " : Inport  Port=3
  Gain1 : Gain  Gain=1/9.81
  Gain2 : Gain  Gain=1/9.81
  Product4 : Product  Inputs=4  SaturateOnIntegerOverflow=on  OutDataTypeStr=Inherit: Same as first input
  Product5 : Product  SaturateOnIntegerOverflow=on  OutDataTypeStr=Inherit: Same as first input
  Sum3 : Sum  Inputs=+-|  SaturateOnIntegerOverflow=on
  Trigonometric Function : Trigonometry  Operator=cos
  We (rad/sec) : Outport  VectorParamsAs1DForOutWhenUnconnected=off
  Ke : Outport  Port=2  VectorParamsAs1DForOutWhenUnconnected=off
  wires:
  "Enc. Angle "/1 -> Trigonometric Function/1
  Trigonometric Function/1 -> Product4/4
  U/1 -> Product4/3
  Gain2/1 -> Ke/1
  "W "/1 -> Sum3/1, Product4/2, Product4/1
  Product5/1 -> Gain2/1
  Sum3/1 -> We (rad/sec)/1, Product5/1, Product5/2
  Gain1/1 -> Sum3/2
  Product4/1 -> Gain1/1
